simulink model "IFOC_BLOCKS"  (R2025a)
settings: Solver=ode4  StartTime=0.0  StopTime=t_stop  FixedStep=h_step  RelTol=1e-3
InitFcn:
  | addpath(fileparts(get_param('IFOC_BLOCKS','FileName'))); bm_drive = 'IFOC'; bm_model = 'IFOC_BLOCKS'; block_model_params;
values from neighbouring files (symbols this model uses):
  Bm = m.B    [block_model_params.m]
  Esw = P.inv.Esw    [block_model_params.m]
  flux_mode_default = c.flux_mode    [block_model_params.m]
  h_step = 5e-6    (= 5e-06)    [block_model_params.m]
  Iref_sw = P.inv.Iref    [block_model_params.m]
  Jm = m.J    [block_model_params.m]
  ke = m.ke    [block_model_params.m]
  kh = m.kh    [block_model_params.m]
  Ki_i = c.Ki_i    [block_model_params.m]
  Ko = c.Ko    [block_model_params.m]
  Kp_i = c.Kp_i    [block_model_params.m]
  Kp_w = c.Kp_w    [block_model_params.m]
  Llr = m.Llr    [block_model_params.m]
  Lls = m.Lls    [block_model_params.m]
  Lm0 = m.Lm0    [block_model_params.m]
  Lm_rated = m.Lm_rated    [block_model_params.m]
  lut_an = P.lut.psi    [block_model_params.m]
  lut_ml = bm_P.lut.psi; end    [block_model_params.m]
  lut_T = P.lut.T(:)'    [block_model_params.m]
  lut_w = P.lut.w(:)'    [block_model_params.m]
  mlp_b1 = double(bm_M.b1(:))    [block_model_params.m]
  mlp_b2 = double(bm_M.b2)    [block_model_params.m]
  mlp_W1 = double(bm_M.W1)    [block_model_params.m]
  mlp_W2 = double(bm_M.W2(:)')    [block_model_params.m]
  mlp_x_mu = double(bm_M.x_mu(:))    [block_model_params.m]
  mlp_x_sd = double(bm_M.x_sd(:))    [block_model_params.m]
  mlp_y_mu = double(bm_M.y_mu)    [block_model_params.m]
  mlp_y_sd = double(bm_M.y_sd)    [block_model_params.m]
  mras_Ki = c.mras_Ki    [block_model_params.m]
  mras_Kp = c.mras_Kp    [block_model_params.m]
  mras_wc = c.mras_wc    [block_model_params.m]
  NT = round(Ts/h)    [block_log_to_thesis.m]    (also in block_model_params.m = round(Ts/h_step))
  pp = m.p    [block_model_params.m]
  psi_k = m.psi_k    [block_model_params.m]
  rad2rpm = 60/(2*pi)    (= 9.54929658551)    [block_model_params.m]
  rce = P.inv.rce    [block_model_params.m]
  rpm2rad = 2*pi/60    (= 0.10471975512)    [block_model_params.m]
  Rr = m.Rr    [block_model_params.m]
  Rs = m.Rs    [block_model_params.m]
  s32 = sqrt(3)/2    [block_model_params.m]
  sat_a = m.sat_a    [block_model_params.m]
  sat_b = m.sat_b    [block_model_params.m]
  sat_on = m.sat_on    [block_model_params.m]
  speed_mode_default = c.speed_mode    [block_model_params.m]
  t_fault = 0.8    [block_model_params.m]
  Te_max = c.Te_max    [block_model_params.m]
  Ts = P.ctrl.Ts    [block_log_to_thesis.m]    (also in block_model_params.m = c.Ts)
  twopi = 2*pi    (= 6.28318530718)    [block_model_params.m]
  Vce0 = P.inv.Vce0    [block_model_params.m]
  Vdc = P.inv.Vdc    [block_model_params.m]
  Vref_sw = P.inv.Vref    [block_model_params.m]
(part 2 of 2)

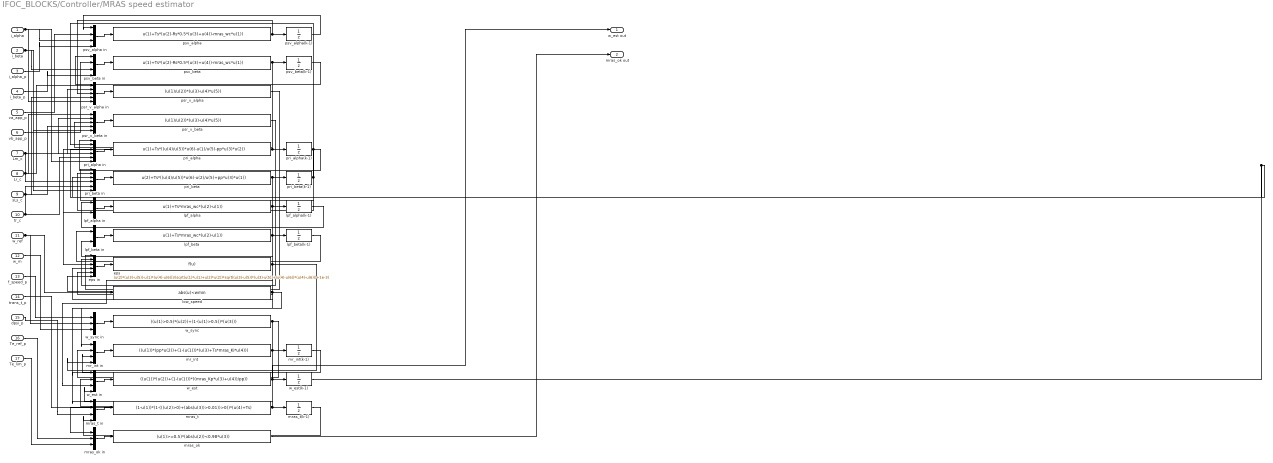
== system IFOC_BLOCKS/Controller/MRAS speed estimator ==
  i_alpha : Inport
  i_beta : Inport  Port=2
  i_alpha_p : Inport  Port=3
  i_beta_p : Inport  Port=4
  va_app_p : Inport  Port=5
  vb_app_p : Inport  Port=6
  Lm_c : Inport  Port=7
  Lr_c : Inport  Port=8
  sLs_c : Inport  Port=9
  tr_c : Inport  Port=10
  w_ref : Inport  Port=11
  w_m : Inport  Port=12
  f_speed_p : Inport  Port=13
  trans_t_p : Inport  Port=14
  dpsi_p : Inport  Port=15
  Te_ref_p : Inport  Port=16
  Te_lim_p : Inport  Port=17
  eps : Fcn  Expr=(u(2)*(u(3)-u(5))-u(1)*(u(4)-u(6)))/(sqrt(u(1)*u(1)+u(2)*u(2))*sqrt((u(3)-u(5))*(u(3)-u(5))+(u(4)-u(6))*(u(4)-u(6)))+1e-3)
  eps in : Mux  Inputs=6
  low_speed : Fcn  Expr=abs(u)<wmin
  lpf_alpha : Fcn  Expr=u(1)+Ts*mras_wc*(u(2)-u(1))
  lpf_alpha in : Mux  Inputs=2
  lpf_alpha(k-1) : UnitDelay  SampleTime=Ts  HasFrameUpgradeWarning=on
  lpf_beta : Fcn  Expr=u(1)+Ts*mras_wc*(u(2)-u(1))
  lpf_beta in : Mux  Inputs=2
  lpf_beta(k-1) : UnitDelay  SampleTime=Ts  HasFrameUpgradeWarning=on
  mr_int : Fcn  Expr=((u(1))*(pp*u(2))+(1-(u(1)))*(u(3)+Ts*mras_Ki*u(4)))
  mr_int in : Mux
  mr_int(k-1) : UnitDelay  SampleTime=Ts  HasFrameUpgradeWarning=on
  mras_ok : Fcn  Expr=(u(1)>=0.5)*(abs(u(2))<0.98*u(3))
  mras_ok in : Mux  Inputs=3
  mras_t : Fcn  Expr=(1-u(1))*(1-(((u(2)>0)+(abs(u(3))>0.01))>0))*(u(4)+Ts)
  mras_t in : Mux
  mras_t(k-1) : UnitDelay  SampleTime=Ts  HasFrameUpgradeWarning=on
  pri_alpha : Fcn  Expr=u(1)+Ts*((u(4)/u(5))*u(6)-u(1)/u(5)-pp*u(3)*u(2))
  pri_alpha in : Mux  Inputs=6
  pri_alpha(k-1) : UnitDelay  SampleTime=Ts  HasFrameUpgradeWarning=on
  pri_beta : Fcn  Expr=u(2)+Ts*((u(4)/u(5))*u(6)-u(2)/u(5)+pp*u(3)*u(1))
  pri_beta in : Mux  Inputs=6
  pri_beta(k-1) : UnitDelay  SampleTime=Ts  HasFrameUpgradeWarning=on
  psr_v_alpha : Fcn  Expr=(u(1)/u(2))*(u(3)-u(4)*u(5))
  psr_v_alpha in : Mux  Inputs=5
  psr_v_beta : Fcn  Expr=(u(1)/u(2))*(u(3)-u(4)*u(5))
  psr_v_beta in : Mux  Inputs=5
  psv_alpha : Fcn  Expr=u(1)+Ts*(u(2)-Rs*0.5*(u(3)+u(4))-mras_wc*u(1))
  psv_alpha in : Mux
  psv_alpha(k-1) : UnitDelay  SampleTime=Ts  HasFrameUpgradeWarning=on
  psv_beta : Fcn  Expr=u(1)+Ts*(u(2)-Rs*0.5*(u(3)+u(4))-mras_wc*u(1))
  psv_beta in : Mux
  psv_beta(k-1) : UnitDelay  SampleTime=Ts  HasFrameUpgradeWarning=on
  w_est : Fcn  Expr=((u(1))*(u(2))+(1-(u(1)))*((mras_Kp*u(3)+u(4))/pp))
  w_est in : Mux
  w_est(k-1) : UnitDelay  SampleTime=Ts  HasFrameUpgradeWarning=on
  w_sync : Fcn  Expr=((u(1)>0.5)*(u(2))+(1-(u(1)>0.5))*(u(3)))
  w_sync in : Mux  Inputs=3
  w_est out : Outport
  mras_ok out : Outport  Port=2
  wires:
  psv_alpha(k-1)/1 -> psv_alpha in/1
  va_app_p/1 -> psv_alpha in/2
  i_alpha/1 -> psv_alpha in/3, psr_v_alpha in/5, pri_alpha in/6
  i_alpha_p/1 -> psv_alpha in/4
  psv_alpha in/1 -> psv_alpha/1
  psv_alpha/1 -> psv_alpha(k-1)/1, psr_v_alpha in/3
  psv_beta(k-1)/1 -> psv_beta in/1
  vb_app_p/1 -> psv_beta in/2
  i_beta/1 -> psv_beta in/3, psr_v_beta in/5, pri_beta in/6
  i_beta_p/1 -> psv_beta in/4
  psv_beta in/1 -> psv_beta/1
  psv_beta/1 -> psv_beta(k-1)/1, psr_v_beta in/3
  Lr_c/1 -> psr_v_alpha in/1, psr_v_beta in/1
  Lm_c/1 -> psr_v_alpha in/2, psr_v_beta in/2, pri_alpha in/4, pri_beta in/4
  sLs_c/1 -> psr_v_alpha in/4, psr_v_beta in/4
  psr_v_alpha in/1 -> psr_v_alpha/1
  psr_v_beta in/1 -> psr_v_beta/1
  pri_alpha(k-1)/1 -> pri_alpha in/1, pri_beta in/1
  pri_beta(k-1)/1 -> pri_alpha in/2, pri_beta in/2
  w_est(k-1)/1 -> pri_alpha in/3, pri_beta in/3
  tr_c/1 -> pri_alpha in/5, pri_beta in/5
  pri_alpha in/1 -> pri_alpha/1
  pri_alpha/1 -> pri_alpha(k-1)/1, lpf_alpha in/2, eps in/3
  pri_beta in/1 -> pri_beta/1
  pri_beta/1 -> pri_beta(k-1)/1, lpf_beta in/2, eps in/4
  lpf_alpha(k-1)/1 -> lpf_alpha in/1
  lpf_alpha in/1 -> lpf_alpha/1
  lpf_alpha/1 -> lpf_alpha(k-1)/1, eps in/5
  lpf_beta(k-1)/1 -> lpf_beta in/1
  lpf_beta in/1 -> lpf_beta/1
  lpf_beta/1 -> lpf_beta(k-1)/1, eps in/6
  psr_v_alpha/1 -> eps in/1
  psr_v_beta/1 -> eps in/2
  eps in/1 -> eps/1
  w_ref/1 -> low_speed/1, w_sync in/2
  f_speed_p/1 -> w_sync in/1
  w_m/1 -> w_sync in/3
  w_sync in/1 -> w_sync/1
  low_speed/1 -> mr_int in/1, w_est in/1, mras_t in/1
  w_sync/1 -> mr_int in/2, w_est in/2
  mr_int(k-1)/1 -> mr_int in/3
  eps/1 -> mr_int in/4, w_est in/3
  mr_int in/1 -> mr_int/1
  mr_int/1 -> mr_int(k-1)/1, w_est in/4
  w_est in/1 -> w_est/1
  w_est/1 -> w_est(k-1)/1, w_est out/1
  trans_t_p/1 -> mras_t in/2
  dpsi_p/1 -> mras_t in/3
  mras_t(k-1)/1 -> mras_t in/4
  mras_t in/1 -> mras_t/1
  mras_t/1 -> mras_t(k-1)/1, mras_ok in/1
  Te_ref_p/1 -> mras_ok in/2
  Te_lim_p/1 -> mras_ok in/3
  mras_ok in/1 -> mras_ok/1
  mras_ok/1 -> mras_ok out/1

== system IFOC_BLOCKS/Controller/Model inductances ==
  psi_ref_p : Inport
  D_c : Fcn  Expr=u(2)*u(3)-u(1)*u(1)
  D_c in : Mux  Inputs=3
  Lm_c : Fcn  Expr=Lm_rated+ctrl_sat*(Lm0/(1+sat_a*((((u)>(0.05))*(u)+((u)<=(0.05))*(0.05))/psi_k)^sat_b)-Lm_rated)
  Lr_c : Fcn  Expr=Llr+u
  Ls_c : Fcn  Expr=Lls+u
  sLs_c : Fcn  Expr=u(2)-u(1)*u(1)/u(3)
  sLs_c in : Mux  Inputs=3
  tr_c : Fcn  Expr=u/Rr
  Lm_c out : Outport
  Ls_c out : Outport  Port=2
  Lr_c out : Outport  Port=3
  sLs_c out : Outport  Port=4
  tr_c out : Outport  Port=5
  D_c out : Outport  Port=6
  wires:
  psi_ref_p/1 -> Lm_c/1
  Lm_c/1 -> Ls_c/1, Lr_c/1, sLs_c in/1, D_c in/1, Lm_c out/1
  Ls_c/1 -> sLs_c in/2, D_c in/2, Ls_c out/1
  Lr_c/1 -> sLs_c in/3, tr_c/1, D_c in/3, Lr_c out/1
  sLs_c in/1 -> sLs_c/1
  D_c in/1 -> D_c/1
  sLs_c/1 -> sLs_c out/1
  tr_c/1 -> tr_c out/1
  D_c/1 -> D_c out/1

== system IFOC_BLOCKS/Controller/Speed controller ==
  w_ref : Inport
  w_u : Inport  Port=2
  Te_lim : Inport  Port=3
  mode : Inport  Port=4
  Te_pi : Fcn  Expr=((((((u(1))>(-u(2)))*(u(1))+((u(1))<=(-u(2)))*(-u(2))))<(u(2)))*((((u(1))>(-u(2)))*(u(1))+((u(1))<=(-u(2)))*(-u(2))))+(((((u(1))>(-u(2)))*(u(1))+((u(1))<=(-u(2)))*(-u(2))))>=(u(2)))*(u(2)))
  Te_pi in : Mux  Inputs=2
  Te_ref : Fcn  Expr=((u(1)>1.5)*(relay_bias+u(2)*relay_T)+(1-(u(1)>1.5))*(u(3)))
  Te_ref in : Mux  Inputs=3
  Te_ref(k-1) : UnitDelay  SampleTime=Ts  HasFrameUpgradeWarning=on
  Te_u : Fcn  Expr=Kp_w*u(1)+u(2)
  Te_u in : Mux  Inputs=2
  e_w : Fcn  Expr=u(1)-u(2)
  e_w in : Mux  Inputs=2
  int_w : Fcn  Expr=((u(1)>1.5)*(u(2))+(1-(u(1)>1.5))*(((((abs(u(3))<=u(4))+(abs(((u(5)>0)-(u(5)<0))-((u(3)>0)-(u(3)<0)))>0.5))>0)*(((((((u(2)+Ts*Ki_w*u(5))>(-u(4)))*(u(2)+Ts*Ki_w*u(5))+((u(2)+Ts*Ki_w*u(5))<=(-u(4)))*(-u(4))))<(u(4)))*((((u(2)+Ts*Ki_w*u(5))>(-u(4)))*(u(2)+Ts*Ki_w*u(5))+((u(2)+Ts*Ki_w*u(5))<=(-u(4)))*(-u(4))))+(((((u(2)+Ts*Ki_w*u(5))>(-u(4)))*(u(2)+Ts*Ki_w*u(5))+((u(2)+Ts*Ki_w*u(5))<=(-u(4)))*(-u(4))))>=(u(4)))*(u(4))))+(1-(((abs(u(3))<=u(4))+(abs(((u(5)>0)-(u(5)<0))-((u(3)>0)-(u(3)<0)))>0.5))>0))*(u(2)))))
  int_w in : Mux  Inputs=5
  int_w(k-1) : UnitDelay  SampleTime=Ts  HasFrameUpgradeWarning=on
  relay : Fcn  Expr=((u(1)>1.5)*(((u(2)>relay_h)*(1)+(1-(u(2)>relay_h))*(((u(2)<-relay_h)*(-1)+(1-(u(2)<-relay_h))*(u(3))))))+(1-(u(1)>1.5))*(u(3)))
  relay in : Mux  Inputs=3
  relay(k-1) : UnitDelay  InitialCondition=1  SampleTime=Ts  HasFrameUpgradeWarning=on
  Te_ref out : Outport
  e_w out : Outport  Port=2
  Te_ref_p out : Outport  Port=3
  wires:
  w_ref/1 -> e_w in/1
  w_u/1 -> e_w in/2
  e_w in/1 -> e_w/1
  mode/1 -> relay in/1, Te_ref in/1, int_w in/1
  e_w/1 -> relay in/2, Te_u in/1, int_w in/5, e_w out/1
  relay(k-1)/1 -> relay in/3
  relay in/1 -> relay/1
  relay/1 -> relay(k-1)/1, Te_ref in/2
  int_w(k-1)/1 -> Te_u in/2, int_w in/2
  Te_u in/1 -> Te_u/1
  Te_u/1 -> Te_pi in/1, int_w in/3
  Te_lim/1 -> Te_pi in/2, int_w in/4
  Te_pi in/1 -> Te_pi/1
  Te_pi/1 -> Te_ref in/3
  Te_ref in/1 -> Te_ref/1
  Te_ref/1 -> Te_ref(k-1)/1, Te_ref out/1
  int_w in/1 -> int_w/1
  int_w/1 -> int_w(k-1)/1
  Te_ref(k-1)/1 -> Te_ref_p out/1

== system IFOC_BLOCKS/Inverter and motor/Core loss ==
  psim_alpha : Inport
  psim_beta : Inport  Port=2
  Pfe : Fcn  Expr=(kh*abs(u(1))+ke*u(1)*u(1))*(u(2)*u(2)+u(3)*u(3))
  Pfe in : Mux  Inputs=3
  angle step : Fcn  Expr=u(1)-u(2)
  angle step in : Mux  Inputs=2
  fe : Fcn  Expr=(u-twopi*floor(u/twopi+0.5))/(twopi*Ts)
  flux angle : Fcn  Expr=atan2(u(2),u(1))
  flux angle in : Mux  Inputs=2
  flux angle(k-1) : UnitDelay  SampleTime=Ts  HasFrameUpgradeWarning=on
  psim_alpha sample : ZeroOrderHold  SampleTime=Ts
  psim_beta sample : ZeroOrderHold  SampleTime=Ts
  Pfe out : Outport
  wires:
  psim_alpha/1 -> psim_alpha sample/1
  psim_beta/1 -> psim_beta sample/1
  psim_alpha sample/1 -> flux angle in/1, Pfe in/2
  psim_beta sample/1 -> flux angle in/2, Pfe in/3
  flux angle in/1 -> flux angle/1
  flux angle/1 -> flux angle(k-1)/1, angle step in/1
  flux angle(k-1)/1 -> angle step in/2
  angle step in/1 -> angle step/1
  angle step/1 -> fe/1
  fe/1 -> Pfe in/1
  Pfe in/1 -> Pfe/1
  Pfe/1 -> Pfe out/1

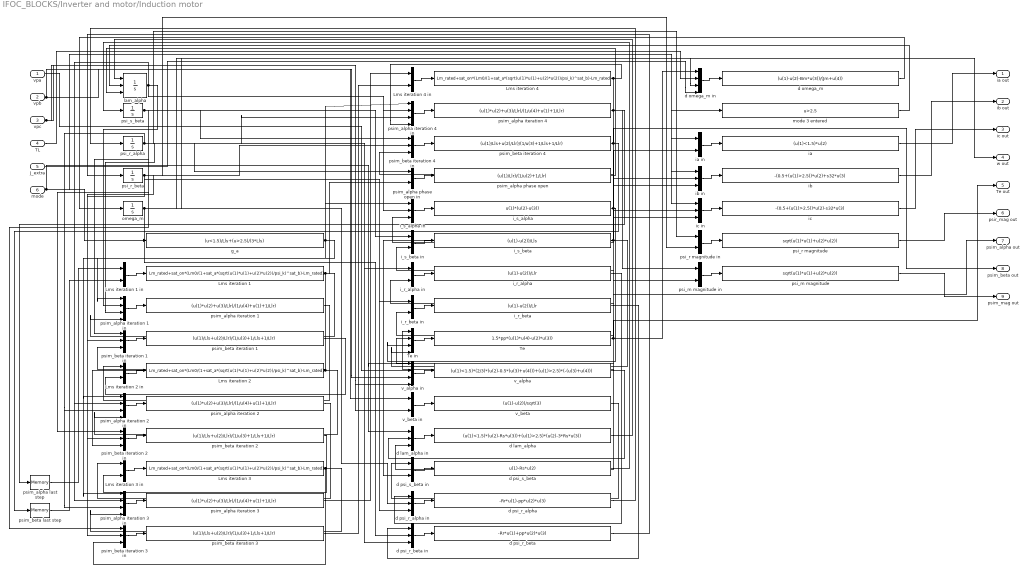
== system IFOC_BLOCKS/Inverter and motor/Induction motor ==
  vpa : Inport
  vpb : Inport  Port=2
  vpc : Inport  Port=3
  TL : Inport  Port=4
  J_extra : Inport  Port=5
  mode : Inport  Port=6
  Lms iteration {1..4} (4 alike) : Fcn  Expr=Lm_rated+sat_on*(Lm0/(1+sat_a*(sqrt(u(1)*u(1)+u(2)*u(2))/psi_k)^sat_b)-Lm_rated)
  Lms iteration 1 in : Mux  Inputs=2
  Lms iteration 2 in : Mux  Inputs=2
  Lms iteration 3 in : Mux  Inputs=2
  Lms iteration 4 in : Mux  Inputs=2
  Te : Fcn  Expr=1.5*pp*(u(1)*u(4)-u(2)*u(3))
  Te in : Mux
  d lam_alpha : Fcn  Expr=(u(1)<1.5)*(u(2)-Rs*u(3))+(u(1)>2.5)*(u(2)-3*Rs*u(3))
  d lam_alpha in : Mux  Inputs=3
  d omega_m : Fcn  Expr=(u(1)-u(2)-Bm*u(3))/(Jm+u(4))
  d omega_m in : Mux
  d psi_r_alpha : Fcn  Expr=-Rr*u(1)-pp*u(2)*u(3)
  d psi_r_alpha in : Mux  Inputs=3
  d psi_r_beta : Fcn  Expr=-Rr*u(1)+pp*u(2)*u(3)
  d psi_r_beta in : Mux  Inputs=3
  d psi_s_beta : Fcn  Expr=u(1)-Rs*u(2)
  d psi_s_beta in : Mux  Inputs=2
  g_a : Fcn  Expr=(u<1.5)/Lls+(u>2.5)/(3*Lls)
  i_r_alpha : Fcn  Expr=(u(1)-u(2))/Llr
  i_r_alpha in : Mux  Inputs=2
  i_r_beta : Fcn  Expr=(u(1)-u(2))/Llr
  i_r_beta in : Mux  Inputs=2
  i_s_alpha : Fcn  Expr=u(1)*(u(2)-u(3))
  i_s_alpha in : Mux  Inputs=3
  i_s_beta : Fcn  Expr=(u(1)-u(2))/Lls
  i_s_beta in : Mux  Inputs=2
  ia : Fcn  Expr=(u(1)<1.5)*u(2)
  ia in : Mux  Inputs=2
  ib : Fcn  Expr=-(0.5+(u(1)>2.5))*u(2)+s32*u(3)
  ib in : Mux  Inputs=3
  ic : Fcn  Expr=-(0.5+(u(1)>2.5))*u(2)-s32*u(3)
  ic in : Mux  Inputs=3
  lam_alpha : Integrator  ExternalReset=rising  InitialConditionSource=external
  mode 3 entered : Fcn  Expr=u>2.5
  omega_m : Integrator
  psi_m magnitude : Fcn  Expr=sqrt(u(1)*u(1)+u(2)*u(2))
  psi_m magnitude in : Mux  Inputs=2
  psi_r magnitude : Fcn  Expr=sqrt(u(1)*u(1)+u(2)*u(2))
  psi_r magnitude in : Mux  Inputs=2
  psi_r_alpha : Integrator
  psi_r_beta : Integrator
  psi_s_beta : Integrator
  psim_alpha iteration {1..4} (4 alike) : Fcn  Expr=(u(1)*u(2)+u(3)/Llr)/(1/u(4)+u(1)+1/Llr)
  psim_alpha iteration 1 in : Mux
  psim_alpha iteration 2 in : Mux
  psim_alpha iteration 3 in : Mux
  psim_alpha iteration 4 in : Mux
  psim_alpha last step : Memory
  psim_alpha phase open : Fcn  Expr=(u(1)/Llr)/(1/u(2)+1/Llr)
  psim_alpha phase open in : Mux  Inputs=2
  psim_beta iteration {1..4} (4 alike) : Fcn  Expr=(u(1)/Lls+u(2)/Llr)/(1/u(3)+1/Lls+1/Llr)
  psim_beta iteration 1 in : Mux  Inputs=3
  psim_beta iteration 2 in : Mux  Inputs=3
  psim_beta iteration 3 in : Mux  Inputs=3
  psim_beta iteration 4 in : Mux  Inputs=3
  psim_beta last step : Memory
  v_alpha : Fcn  Expr=(u(1)<1.5)*(2/3)*(u(2)-0.5*(u(3)+u(4)))+(u(1)>2.5)*(-(u(3)+u(4)))
  v_alpha in : Mux
  v_beta : Fcn  Expr=(u(1)-u(2))/sqrt(3)
  v_beta in : Mux  Inputs=2
  ia out : Outport
  ib out : Outport  Port=2
  ic out : Outport  Port=3
  w out : Outport  Port=4
  Te out : Outport  Port=5
  psir_mag out : Outport  Port=6
  psim_alpha out : Outport  Port=7
  psim_beta out : Outport  Port=8
  psim_mag out : Outport  Port=9
  wires:
  mode/1 -> g_a/1, v_alpha in/1, d lam_alpha in/1, mode 3 entered/1, ia in/1, ib in/1, ic in/1
  psim_alpha last step/1 -> Lms iteration 1 in/1
  psim_beta last step/1 -> Lms iteration 1 in/2
  Lms iteration 1 in/1 -> Lms iteration 1/1
  g_a/1 -> psim_alpha iteration 1 in/1, psim_alpha iteration 2 in/1, psim_alpha iteration 3 in/1, psim_alpha iteration 4 in/1, i_s_alpha in/1
  lam_alpha/1 -> psim_alpha iteration 1 in/2, psim_alpha iteration 2 in/2, psim_alpha iteration 3 in/2, psim_alpha iteration 4 in/2, i_s_alpha in/2
  psi_r_alpha/1 -> psim_alpha iteration 1 in/3, psim_alpha iteration 2 in/3, psim_alpha iteration 3 in/3, psim_alpha iteration 4 in/3, psim_alpha phase open in/1, i_r_alpha in/1, d psi_r_beta in/3, psi_r magnitude in/1
  Lms iteration 1/1 -> psim_alpha iteration 1 in/4, psim_beta iteration 1 in/3, psim_alpha phase open in/2
  psim_alpha iteration 1 in/1 -> psim_alpha iteration 1/1
  psi_s_beta/1 -> psim_beta iteration 1 in/1, psim_beta iteration 2 in/1, psim_beta iteration 3 in/1, psim_beta iteration 4 in/1, i_s_beta in/1
  psi_r_beta/1 -> psim_beta iteration 1 in/2, psim_beta iteration 2 in/2, psim_beta iteration 3 in/2, psim_beta iteration 4 in/2, i_r_beta in/1, d psi_r_alpha in/3, psi_r magnitude in/2
  psim_beta iteration 1 in/1 -> psim_beta iteration 1/1
  psim_alpha iteration 1/1 -> Lms iteration 2 in/1
  psim_beta iteration 1/1 -> Lms iteration 2 in/2
  Lms iteration 2 in/1 -> Lms iteration 2/1
  Lms iteration 2/1 -> psim_alpha iteration 2 in/4, psim_beta iteration 2 in/3
  psim_alpha iteration 2 in/1 -> psim_alpha iteration 2/1
  psim_beta iteration 2 in/1 -> psim_beta iteration 2/1
  psim_alpha iteration 2/1 -> Lms iteration 3 in/1
  psim_beta iteration 2/1 -> Lms iteration 3 in/2
  Lms iteration 3 in/1 -> Lms iteration 3/1
  Lms iteration 3/1 -> psim_alpha iteration 3 in/4, psim_beta iteration 3 in/3
  psim_alpha iteration 3 in/1 -> psim_alpha iteration 3/1
  psim_beta iteration 3 in/1 -> psim_beta iteration 3/1
  psim_alpha iteration 3/1 -> Lms iteration 4 in/1
  psim_beta iteration 3/1 -> Lms iteration 4 in/2
  Lms iteration 4 in/1 -> Lms iteration 4/1
  Lms iteration 4/1 -> psim_alpha iteration 4 in/4, psim_beta iteration 4 in/3
  psim_alpha iteration 4 in/1 -> psim_alpha iteration 4/1
  psim_beta iteration 4 in/1 -> psim_beta iteration 4/1
  psim_alpha iteration 4/1 -> psim_alpha last step/1, i_s_alpha in/3, i_r_alpha in/2, Te in/1, psi_m magnitude in/1, psim_alpha out/1
  psim_beta iteration 4/1 -> psim_beta last step/1, i_s_beta in/2, i_r_beta in/2, Te in/2, psi_m magnitude in/2, psim_beta out/1
  psim_alpha phase open in/1 -> psim_alpha phase open/1
  i_s_alpha in/1 -> i_s_alpha/1
  i_s_beta in/1 -> i_s_beta/1
  i_r_alpha in/1 -> i_r_alpha/1
  i_r_beta in/1 -> i_r_beta/1
  i_s_alpha/1 -> Te in/3, d lam_alpha in/3, ia in/2, ib in/2, ic in/2
  i_s_beta/1 -> Te in/4, d psi_s_beta in/2, ib in/3, ic in/3
  Te in/1 -> Te/1
  vpa/1 -> v_alpha in/2
  vpb/1 -> v_alpha in/3, v_beta in/1
  vpc/1 -> v_alpha in/4, v_beta in/2
  v_alpha in/1 -> v_alpha/1
  v_beta in/1 -> v_beta/1
  v_alpha/1 -> d lam_alpha in/2
  d lam_alpha in/1 -> d lam_alpha/1
  v_beta/1 -> d psi_s_beta in/1
  d psi_s_beta in/1 -> d psi_s_beta/1
  i_r_alpha/1 -> d psi_r_alpha in/1
  omega_m/1 -> d psi_r_alpha in/2, d psi_r_beta in/2, d omega_m in/3, w out/1
  d psi_r_alpha in/1 -> d psi_r_alpha/1
  i_r_beta/1 -> d psi_r_beta in/1
  d psi_r_beta in/1 -> d psi_r_beta/1
  Te/1 -> d omega_m in/1, Te out/1
  TL/1 -> d omega_m in/2
  J_extra/1 -> d omega_m in/4
  d omega_m in/1 -> d omega_m/1
  d lam_alpha/1 -> lam_alpha/1
  mode 3 entered/1 -> lam_alpha/2
  psim_alpha phase open/1 -> lam_alpha/3
  d psi_s_beta/1 -> psi_s_beta/1
  d psi_r_alpha/1 -> psi_r_alpha/1
  d psi_r_beta/1 -> psi_r_beta/1
  d omega_m/1 -> omega_m/1
  ia in/1 -> ia/1
  ib in/1 -> ib/1
  ic in/1 -> ic/1
  psi_r magnitude in/1 -> psi_r magnitude/1
  psi_m magnitude in/1 -> psi_m magnitude/1
  ia/1 -> ia out/1
  ib/1 -> ib out/1
  ic/1 -> ic out/1
  psi_r magnitude/1 -> psir_mag out/1
  psi_m magnitude/1 -> psim_mag out/1

== system IFOC_BLOCKS/Inverter and motor/Inverter losses ==
  vpa : Inport
  vpb : Inport  Port=2
  vpc : Inport  Port=3
  ia : Inport  Port=4
  ib : Inport  Port=5
  ic : Inport  Port=6
  trans_a : Inport  Port=7
  trans_b : Inport  Port=8
  trans_c : Inport  Port=9
  Currents at step start : ZeroOrderHold  SampleTime=h_step
  Currents mux : Mux  Inputs=3
  Inverter mux : Mux  Inputs=9
  Pcond : Fcn  Expr=Vce0*(abs(u(4))+abs(u(5))+abs(u(6)))+rce*(u(4)*u(4)+u(5)*u(5)+u(6)*u(6))
  Pel : Fcn  Expr=u(1)*u(4)+u(2)*u(5)+u(3)*u(6)
  Psw : Fcn  Expr=Esw*(Vdc/Vref_sw)/Iref_sw*(u(4)*abs(u(1))+u(5)*abs(u(2))+u(6)*abs(u(3)))/h_step
  Switching mux : Mux  Inputs=2
  Transition count : Fcn  Expr=u(7)+u(8)+u(9)
  Transitions mux : Mux  Inputs=3
  Pel out : Outport
  Pcond out : Outport  Port=2
  Psw out : Outport  Port=3
  transitions out : Outport  Port=4
  wires:
  vpa/1 -> Inverter mux/1
  vpb/1 -> Inverter mux/2
  vpc/1 -> Inverter mux/3
  ia/1 -> Inverter mux/4, Currents mux/1
  ib/1 -> Inverter mux/5, Currents mux/2
  ic/1 -> Inverter mux/6, Currents mux/3
  trans_a/1 -> Inverter mux/7, Transitions mux/1
  trans_b/1 -> Inverter mux/8, Transitions mux/2
  trans_c/1 -> Inverter mux/9, Transitions mux/3
  Currents mux/1 -> Currents at step start/1
  Currents at step start/1 -> Switching mux/1
  Transitions mux/1 -> Switching mux/2
  Switching mux/1 -> Psw/1
  Inverter mux/1 -> Pel/1, Pcond/1, Transition count/1
  Pel/1 -> Pel out/1
  Pcond/1 -> Pcond out/1
  Psw/1 -> Psw out/1
  Transition count/1 -> transitions out/1

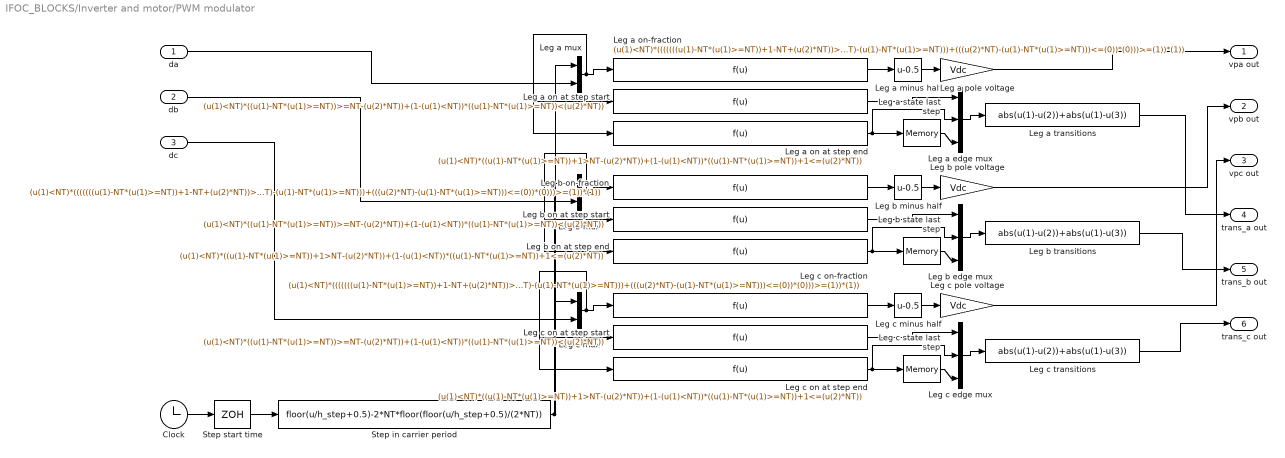
== system IFOC_BLOCKS/Inverter and motor/PWM modulator ==
  da : Inport
  db : Inport  Port=2
  dc : Inport  Port=3
  Clock : Clock
  Leg a edge mux : Mux  Inputs=3
  Leg a minus half : Bias  Bias=-0.5  SaturateOnIntegerOverflow=off
  Leg a mux : Mux  Inputs=2
  Leg a on at step end : Fcn  Expr=(u(1)<NT)*((u(1)-NT*(u(1)>=NT))+1>NT-(u(2)*NT))+(1-(u(1)<NT))*((u(1)-NT*(u(1)>=NT))+1<=(u(2)*NT))
  Leg a on at step start : Fcn  Expr=(u(1)<NT)*((u(1)-NT*(u(1)>=NT))>=NT-(u(2)*NT))+(1-(u(1)<NT))*((u(1)-NT*(u(1)>=NT))<(u(2)*NT))
  Leg a on-fraction : Fcn  Expr=(u(1)<NT)*(((((((u(1)-NT*(u(1)>=NT))+1-NT+(u(2)*NT))>(0))*((u(1)-NT*(u(1)>=NT))+1-NT+(u(2)*NT))+(((u(1)-NT*(u(1)>=NT))+1-NT+(u(2)*NT))<=(0))*(0)))<(1))*(((((u(1)-NT*(u(1)>=NT))+1-NT+(u(2)*NT))>(0))*((u(1)-NT*(u(1)>=NT))+1-NT+(u(2)*NT))+(((u(1)-NT*(u(1)>=NT))+1-NT+(u(2)*NT))<=(0))*(0)))+((((((u(1)-NT*(u(1)>=NT))+1-NT+(u(2)*NT))>(0))*((u(1)-NT*(u(1)>=NT))+1-NT+(u(2)*NT))+(((u(1)-NT*(u(1)>=NT))+1-NT+(u(2)*NT))<=(0))*(0)))>=(1))*(1))+(1-(u(1)<NT))*(((((((u(2)*NT)-(u(1)-NT*(u(1)>=NT)))>(0))*((u(2)*NT)-(u(1)-NT*(u(1)>=NT)))+(((u(2)*NT)-(u(1)-NT*(u(1)>=NT)))<=(0))*(0)))<(1))*(((((u(2)*NT)-(u(1)-NT*(u(1)>=NT)))>(0))*((u(2)*NT)-(u(1)-NT*(u(1)>=NT)))+(((u(2)*NT)-(u(1)-NT*(u(1)>=NT)))<=(0))*(0)))+((((((u(2)*NT)-(u(1)-NT*(u(1)>=NT)))>(0))*((u(2)*NT)-(u(1)-NT*(u(1)>=NT)))+(((u(2)*NT)-(u(1)-NT*(u(1)>=NT)))<=(0))*(0)))>=(1))*(1))
  Leg a pole voltage : Gain  Gain=Vdc
  Leg a state last step : Memory
  Leg a transitions : Fcn  Expr=abs(u(1)-u(2))+abs(u(1)-u(3))
  Leg b edge mux : Mux  Inputs=3
  Leg b minus half : Bias  Bias=-0.5  SaturateOnIntegerOverflow=off
  Leg b mux : Mux  Inputs=2
  Leg b on at step end : Fcn  Expr=(u(1)<NT)*((u(1)-NT*(u(1)>=NT))+1>NT-(u(2)*NT))+(1-(u(1)<NT))*((u(1)-NT*(u(1)>=NT))+1<=(u(2)*NT))
  Leg b on at step start : Fcn  Expr=(u(1)<NT)*((u(1)-NT*(u(1)>=NT))>=NT-(u(2)*NT))+(1-(u(1)<NT))*((u(1)-NT*(u(1)>=NT))<(u(2)*NT))
  Leg b on-fraction : Fcn  Expr=(u(1)<NT)*(((((((u(1)-NT*(u(1)>=NT))+1-NT+(u(2)*NT))>(0))*((u(1)-NT*(u(1)>=NT))+1-NT+(u(2)*NT))+(((u(1)-NT*(u(1)>=NT))+1-NT+(u(2)*NT))<=(0))*(0)))<(1))*(((((u(1)-NT*(u(1)>=NT))+1-NT+(u(2)*NT))>(0))*((u(1)-NT*(u(1)>=NT))+1-NT+(u(2)*NT))+(((u(1)-NT*(u(1)>=NT))+1-NT+(u(2)*NT))<=(0))*(0)))+((((((u(1)-NT*(u(1)>=NT))+1-NT+(u(2)*NT))>(0))*((u(1)-NT*(u(1)>=NT))+1-NT+(u(2)*NT))+(((u(1)-NT*(u(1)>=NT))+1-NT+(u(2)*NT))<=(0))*(0)))>=(1))*(1))+(1-(u(1)<NT))*(((((((u(2)*NT)-(u(1)-NT*(u(1)>=NT)))>(0))*((u(2)*NT)-(u(1)-NT*(u(1)>=NT)))+(((u(2)*NT)-(u(1)-NT*(u(1)>=NT)))<=(0))*(0)))<(1))*(((((u(2)*NT)-(u(1)-NT*(u(1)>=NT)))>(0))*((u(2)*NT)-(u(1)-NT*(u(1)>=NT)))+(((u(2)*NT)-(u(1)-NT*(u(1)>=NT)))<=(0))*(0)))+((((((u(2)*NT)-(u(1)-NT*(u(1)>=NT)))>(0))*((u(2)*NT)-(u(1)-NT*(u(1)>=NT)))+(((u(2)*NT)-(u(1)-NT*(u(1)>=NT)))<=(0))*(0)))>=(1))*(1))
  Leg b pole voltage : Gain  Gain=Vdc
  Leg b state last step : Memory
  Leg b transitions : Fcn  Expr=abs(u(1)-u(2))+abs(u(1)-u(3))
  Leg c edge mux : Mux  Inputs=3
  Leg c minus half : Bias  Bias=-0.5  SaturateOnIntegerOverflow=off
  Leg c mux : Mux  Inputs=2
  Leg c on at step end : Fcn  Expr=(u(1)<NT)*((u(1)-NT*(u(1)>=NT))+1>NT-(u(2)*NT))+(1-(u(1)<NT))*((u(1)-NT*(u(1)>=NT))+1<=(u(2)*NT))
  Leg c on at step start : Fcn  Expr=(u(1)<NT)*((u(1)-NT*(u(1)>=NT))>=NT-(u(2)*NT))+(1-(u(1)<NT))*((u(1)-NT*(u(1)>=NT))<(u(2)*NT))
  Leg c on-fraction : Fcn  Expr=(u(1)<NT)*(((((((u(1)-NT*(u(1)>=NT))+1-NT+(u(2)*NT))>(0))*((u(1)-NT*(u(1)>=NT))+1-NT+(u(2)*NT))+(((u(1)-NT*(u(1)>=NT))+1-NT+(u(2)*NT))<=(0))*(0)))<(1))*(((((u(1)-NT*(u(1)>=NT))+1-NT+(u(2)*NT))>(0))*((u(1)-NT*(u(1)>=NT))+1-NT+(u(2)*NT))+(((u(1)-NT*(u(1)>=NT))+1-NT+(u(2)*NT))<=(0))*(0)))+((((((u(1)-NT*(u(1)>=NT))+1-NT+(u(2)*NT))>(0))*((u(1)-NT*(u(1)>=NT))+1-NT+(u(2)*NT))+(((u(1)-NT*(u(1)>=NT))+1-NT+(u(2)*NT))<=(0))*(0)))>=(1))*(1))+(1-(u(1)<NT))*(((((((u(2)*NT)-(u(1)-NT*(u(1)>=NT)))>(0))*((u(2)*NT)-(u(1)-NT*(u(1)>=NT)))+(((u(2)*NT)-(u(1)-NT*(u(1)>=NT)))<=(0))*(0)))<(1))*(((((u(2)*NT)-(u(1)-NT*(u(1)>=NT)))>(0))*((u(2)*NT)-(u(1)-NT*(u(1)>=NT)))+(((u(2)*NT)-(u(1)-NT*(u(1)>=NT)))<=(0))*(0)))+((((((u(2)*NT)-(u(1)-NT*(u(1)>=NT)))>(0))*((u(2)*NT)-(u(1)-NT*(u(1)>=NT)))+(((u(2)*NT)-(u(1)-NT*(u(1)>=NT)))<=(0))*(0)))>=(1))*(1))
  Leg c pole voltage : Gain  Gain=Vdc
  Leg c state last step : Memory
  Leg c transitions : Fcn  Expr=abs(u(1)-u(2))+abs(u(1)-u(3))
  Step in carrier period : Fcn  Expr=floor(u/h_step+0.5)-2*NT*floor(floor(u/h_step+0.5)/(2*NT))
  Step start time : ZeroOrderHold  SampleTime=h_step
  vpa out : Outport
  vpb out : Outport  Port=2
  vpc out : Outport  Port=3
  trans_a out : Outport  Port=4
  trans_b out : Outport  Port=5
  trans_c out : Outport  Port=6
  wires:
  Clock/1 -> Step start time/1
  Step start time/1 -> Step in carrier period/1
  Step in carrier period/1 -> Leg a mux/1, Leg b mux/1, Leg c mux/1
  da/1 -> Leg a mux/2
  Leg a mux/1 -> Leg a on-fraction/1, Leg a on at step start/1, Leg a on at step end/1
  Leg a on at step end/1 -> Leg a state last step/1, Leg a edge mux/2
  Leg a on at step start/1 -> Leg a edge mux/1
  Leg a state last step/1 -> Leg a edge mux/3
  Leg a edge mux/1 -> Leg a transitions/1
  Leg a on-fraction/1 -> Leg a minus half/1
  Leg a minus half/1 -> Leg a pole voltage/1
  Leg a pole voltage/1 -> vpa out/1
  Leg a transitions/1 -> trans_a out/1
  db/1 -> Leg b mux/2
  Leg b mux/1 -> Leg b on-fraction/1, Leg b on at step start/1, Leg b on at step end/1
  Leg b on at step end/1 -> Leg b state last step/1, Leg b edge mux/2
  Leg b on at step start/1 -> Leg b edge mux/1
  Leg b state last step/1 -> Leg b edge mux/3
  Leg b edge mux/1 -> Leg b transitions/1
  Leg b on-fraction/1 -> Leg b minus half/1
  Leg b minus half/1 -> Leg b pole voltage/1
  Leg b pole voltage/1 -> vpb out/1
  Leg b transitions/1 -> trans_b out/1
  dc/1 -> Leg c mux/2
  Leg c mux/1 -> Leg c on-fraction/1, Leg c on at step start/1, Leg c on at step end/1
  Leg c on at step end/1 -> Leg c state last step/1, Leg c edge mux/2
  Leg c on at step start/1 -> Leg c edge mux/1
  Leg c state last step/1 -> Leg c edge mux/3
  Leg c edge mux/1 -> Leg c transitions/1
  Leg c on-fraction/1 -> Leg c minus half/1
  Leg c minus half/1 -> Leg c pole voltage/1
  Leg c pole voltage/1 -> vpc out/1
  Leg c transitions/1 -> trans_c out/1

== system IFOC_BLOCKS/Controller/Flux reference/MLP network ==
  w : Inport
  T : Inport  Port=2
  Centre : Sum  Inputs=+-
  De-normalise : Sum
  Hidden sum : Sum
  Input mux : Mux  Inputs=2
  Normalise : Gain  Gain=1./mlp_x_sd
  Output sum : Sum
  W1 : Gain  Gain=mlp_W1  Multiplication=Matrix(K*u)
  W2 : Gain  Gain=mlp_W2  Multiplication=Matrix(K*u)
  b1 : Constant  Value=mlp_b1
  b2 : Constant  Value=mlp_b2
  tanh : Trigonometry  Operator=tanh
  x_mu : Constant  Value=mlp_x_mu
  y_mu : Constant  Value=mlp_y_mu
  y_sd : Gain  Gain=mlp_y_sd
  psi out : Outport
  wires:
  w/1 -> Input mux/1
  T/1 -> Input mux/2
  Input mux/1 -> Centre/1
  x_mu/1 -> Centre/2
  Centre/1 -> Normalise/1
  Normalise/1 -> W1/1
  W1/1 -> Hidden sum/1
  b1/1 -> Hidden sum/2
  Hidden sum/1 -> tanh/1
  tanh/1 -> W2/1
  W2/1 -> Output sum/1
  b2/1 -> Output sum/2
  Output sum/1 -> y_sd/1
  y_sd/1 -> De-normalise/1
  y_mu/1 -> De-normalise/2
  De-normalise/1 -> psi out/1
